simulink model "WBR_Simulator"  (R2023b)
settings: Solver=FixedStepAuto  StartTime=0.0  StopTime=60  FixedStep=0.001  MaxStep=0.001
undefined symbols (not defined in the file or in its folder): DiscIntNeverNeededParam, magnitude, robot_stats, SIMPARAM, X, Y, Z
libraries: sm_lib x73, nesl_utility x50, simulink x17, slpidlib x6, dsparch4 x2
(part 2 of 7)

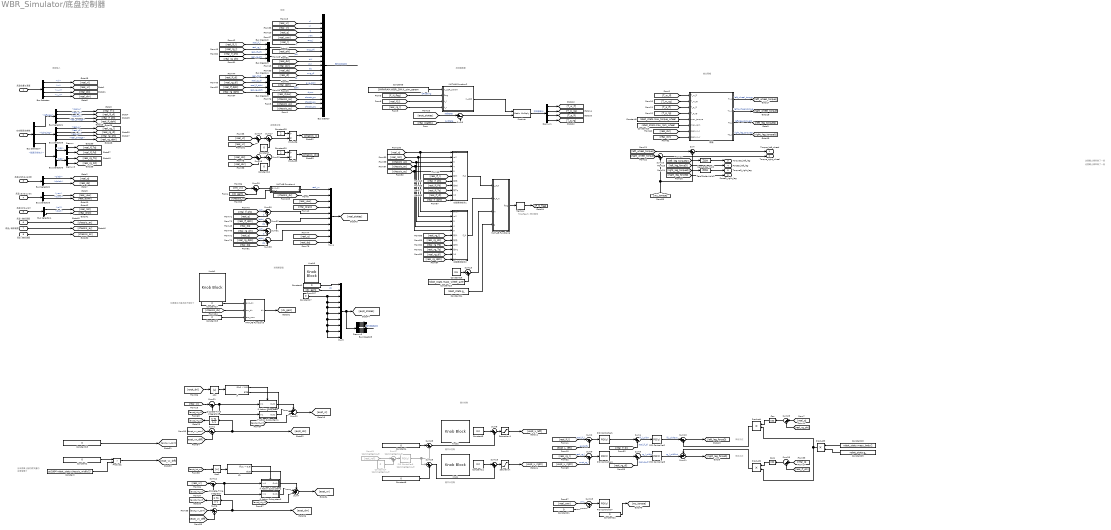
== system WBR_Simulator/底盘控制器 ==
  note: 参数输入
  note: F_N_flag为1表示离地
  note: 加速度过大基本就不受控了
  note: 应该再算上腿的劈叉量的
      | 这里偷懒了
  note: 腿齐长控制
  note: 伸出为正
  note: 伸出为正
  note: 这里截止频率除了一倍
  note: 这里截止频率除了一倍
  note: 腿齐长控制
  note: 装载真实值
  note: 装载期望值
  note: 观测
  note: 腿长控制
  note: 控制器解算
  note: 输出限幅
  底盘位置&速度 : Inport
  左右腿姿态参数 : Inport  Port=2
  底盘pitch&wpitch : Inport  Port=3
  底盘yaw&wyaw : Inport  Port=4
  底盘roll&wroll : Inport  Port=5
  底盘x轴加速度 : Inport  Port=6
  底盘y轴加速度 : Inport  Port=7
  底盘z轴加速度 : Inport  Port=8
  Abs : Abs  SaturateOnIntegerOverflow=off
  Abs1 : Abs  SaturateOnIntegerOverflow=off
  Bus Creator : BusCreator  Inputs=19
  Bus Creator{2..5} (4 alike) : BusCreator  Inputs=2
  Bus Creator8 : BusCreator  Inputs=10
  Bus Selector : BusSelector  OutputSignals=xl,xr,v_xl,v_xr
  Bus Selector1 : BusSelector  OutputSignals=real_L,real_dl,real_phi,real_omega
  Bus Selector2 : BusSelector  OutputSignals=pitch,dpitch
  Bus Selector3 : BusSelector  OutputSignals=yaw,dyaw
  Bus Selector4 : BusSelector  OutputSignals=roll,droll
  Bus Selector5 : BusSelector  OutputSignals=real_L,real_dl,real_phi,real_omega
  Bus Selector6 : BusSelector  OutputSignals=左腿,右腿
  Bus Selector7 : BusSelector  OutputSignals=left_leg,right_leg,腿真实有效力
  Constant : Constant  Value=pi/180*(robot_stats.chassis_width/2)
  Constant{1..2,4,7,12,15,17,21..22} (9 alike) : Constant  Value=0
  Constant10 : Constant  Value=robot_stats.max_rpm_wheel
  Constant11 : Constant  Value=0.2
  Constant14 : Constant  Commented=on  Value=0
  Constant16 : Constant  Value=0.5
  Constant18 : Constant  Value=robot_stats.mass_body/2
  Constant{19..20,27..28} (4 alike) : Constant  Value=2
  Constant23 : Constant  Value=robot_stats.mass_wheel_aver
  Constant24 : Constant  Value=robot_stats.g_
  Constant25 : Constant  Value=robot_stats.g_
  Constant3 : Constant  Value=0.2
  Constant5 : Constant  Value=SIMPARAM.WBR_SIM.K_sim_param
  Constant8 : Constant  Value=0  VectorParams1D=off
  Constant9 : Constant  Value=robot_stats.max_torque_wheel
  Cos : Trigonometry  Operator=cos
  Cos1 : Trigonometry  Operator=cos
  Demux : Demux  Outputs=2
  Demux1 : Demux
  Demux3 : Demux  Outputs=2
  Demux6 : Demux  Outputs=10
  Discrete-Time Integrator : DiscreteIntegrator  SampleTime=-1  ICPrevOutput=DiscIntNeverNeededParam  ICPrevScaledInput=DiscIntNeverNeededParam
  Discrete-Time Integrator1 : DiscreteIntegrator  SampleTime=-1  ICPrevOutput=DiscIntNeverNeededParam  ICPrevScaledInput=DiscIntNeverNeededParam
  From61 : From  Commented=on  GotoTag=real_roll
  If : If  IfExpression=u1 < 0.5
  If Action Subsystem : Subsystem  TreatAsAtomicUnit=on
  If Action Subsystem1 : Subsystem  TreatAsAtomicUnit=on
  If Action Subsystem2 : Subsystem  TreatAsAtomicUnit=on
  If Action Subsystem3 : Subsystem  TreatAsAtomicUnit=on
  If1 : If  IfExpression=u1 < 0.5
  Knob : KnobBlock  ScaleMin=-1  ScaleMax=1
  Knob1 : KnobBlock
  Knob2 : KnobBlock  ScaleMin=-1  ScaleMax=1
  Knob3 : KnobBlock
  MATLAB Function2 : MATLAB Function  TreatAsAtomicUnit=on
  MATLAB Function4 : MATLAB Function  TreatAsAtomicUnit=on
  MATLAB Function5 : MATLAB Function  TreatAsAtomicUnit=on
  MATLAB Function6 : MATLAB Function  TreatAsAtomicUnit=on
  Memory : Memory
  Mux4 : Mux  Inputs=10
  Mux5 : Mux  Inputs=10
  PID Controller1 : slpidlib/PID Controller  Controller=PID  Form=Parallel  TimeDomain=Discrete-time  UseExternalTs=off  SampleTime=-1  IntegratorMethod=Forward Euler  FilterMethod=Forward Euler  ControllerParametersSource=internal  P=8  I=0  UseKiTs=on  D=0.1  N=200  UseFilter=on  TunerSelectOption=Transfer Function Based (PID Tuner App)  InitialConditionSource=internal  InitialConditionForIntegrator=0  InitialConditionForFilter=0  DifferentiatorICPrevScaledInput=0  ExternalReset=none  TrackingMode=off  Kt=1  LimitOutput=off  SatLimitsSource=internal  UpperSaturationLimit=inf  LowerSaturationLimit=-inf  LinearizeAsGain=on  AntiWindupMode=none  Kb=1  LimitIntegrator=off  UpperIntegratorSaturationLimit=inf  LowerIntegratorSaturationLimit=-inf  POutMin=[]  POutMax=[]  IOutMin=[]  IOutMax=[]  DOutMin=[]  DOutMax=[]  NOutMin=[]  NOutMax=[]  SumOutMin=[]  SumOutMax=[]  SaturationOutMin=[]  SaturationOutMax=[]  PParamMin=[]  PParamMax=[]  IParamMin=[]  IParamMax=[]  DParamMin=[]  DParamMax=[]  NParamMin=[]  NParamMax=[]  KbParamMin=[]  KbParamMax=[]  KtParamMin=[]  KtParamMax=[]  KbOutMin=[]  KbOutMax=[]  KtOutMin=[]  KtOutMax=[]  IntegratorOutMin=[]  IntegratorOutMax=[]  FilterOutMin=[]  FilterOutMax=[]  SumI1OutMin=[]  SumI1OutMax=[]  SumI2OutMin=[]  SumI2OutMax=[]  SumI3OutMin=[]  SumI3OutMax=[]  SumI4OutMin=[]  SumI4OutMax=[]  SumDOutMin=[]  SumDOutMax=[]  DifferentiatorOutMin=[]  DifferentiatorOutMax=[]  FilterDiffOutCoefMin=[]  FilterDiffOutCoefMax=[]  ReciprocalOutMin=[]  ReciprocalOutMax=[]  SumDenOutMin=[]  SumDenOutMax=[]  SumNumOutMin=[]  SumNumOutMax=[]  DivideOutMin=[]  DivideOutMax=[]  UdiffTsProdOutMin=[]  UdiffTsProdOutMax=[]  NTsProdOutMin=[]  NTsProdOutMax=[]  UintegralTsProdOutMin=[]  UintegralTsProdOutMax=[]  UngainTsProdOutMin=[]  UngainTsProdOutMax=[]  ClampingZeroOutDataTypeStr=Inherit: Inherit via back propagation  ClampingZeroOutMin=[]  ClampingZeroOutMax=[]  FilterDenConstantOutDataTypeStr=Inherit: Inherit via back propagation  FilterDenConstantOutMin=[]  FilterDenConstantOutMax=[]  PCopyOutDataTypeStr=Inherit: Inherit via back propagation  PCopyOutMin=[]  PCopyOutMax=[]  NCopyOutDataTypeStr=Inherit: Inherit via back propagation  NCopyOutMin=[]  NCopyOutMax=[]  IntegratorContinuousStateAttributes=''  IntegratorStateMustResolveToSignalObject=off  IntegratorRTWStateStorageClass=Auto  FilterContinuousStateAttributes=''  FilterStateMustResolveToSignalObject=off  FilterRTWStateStorageClass=Auto  ParallelPVariant=InternalParameters  IdealPVariant=Disabled  IVariant=InternalParameters  DVariant=InternalParameters  IntegratorVariant=Discrete  SatVariant=Disabled  AWVariant=Passthrough  PCopyVariant=Disabled  TRVariant=Disabled  FdbkBlocksVariant=Forward  IdealPFdbkVariant=Disabled  SatFdbkVariant=Disabled  DerivativeFilterVariant=ForwardEulerFilter  NVariant=InternalParameters  NCopyVariant=Disabled  FilterICVariant=InternalICsFilter  IntegratorICVariant=InternalICs  ExternalResetVariant=Disabled  TRSumVariant=Passthrough  SumFdbkVariant=Disabled  SumVariant=Sum_PID  TsampFilterVariant=InternalTs  TsampNgainVariant=Passthrough  TsampIntegralVariant=Disabled_SignalSpec  ExternalSaturationOutDataTypeStr=Inherit: Same as second input
  PID Controller2 : slpidlib/PID Controller  Controller=PID  Form=Parallel  TimeDomain=Discrete-time  UseExternalTs=off  SampleTime=-1  IntegratorMethod=Forward Euler  FilterMethod=Forward Euler  ControllerParametersSource=internal  P=50  I=0  UseKiTs=off  D=0.1  N=100  UseFilter=on  TunerSelectOption=Transfer Function Based (PID Tuner App)  InitialConditionSource=internal  InitialConditionForIntegrator=0  InitialConditionForFilter=0  DifferentiatorICPrevScaledInput=0  ExternalReset=none  TrackingMode=off  Kt=1  LimitOutput=off  SatLimitsSource=internal  UpperSaturationLimit=800  LowerSaturationLimit=-800  LinearizeAsGain=on  AntiWindupMode=none  Kb=1  LimitIntegrator=off  UpperIntegratorSaturationLimit=inf  LowerIntegratorSaturationLimit=-inf  POutMin=[]  POutMax=[]  IOutMin=[]  IOutMax=[]  DOutMin=[]  DOutMax=[]  NOutMin=[]  NOutMax=[]  SumOutMin=[]  SumOutMax=[]  SaturationOutMin=[]  SaturationOutMax=[]  PParamMin=[]  PParamMax=[]  IParamMin=[]  IParamMax=[]  DParamMin=[]  DParamMax=[]  NParamMin=[]  NParamMax=[]  KbParamMin=[]  KbParamMax=[]  KtParamMin=[]  KtParamMax=[]  KbOutMin=[]  KbOutMax=[]  KtOutMin=[]  KtOutMax=[]  IntegratorOutMin=[]  IntegratorOutMax=[]  FilterOutMin=[]  FilterOutMax=[]  SumI1OutMin=[]  SumI1OutMax=[]  SumI2OutMin=[]  SumI2OutMax=[]  SumI3OutMin=[]  SumI3OutMax=[]  SumI4OutMin=[]  SumI4OutMax=[]  SumDOutMin=[]  SumDOutMax=[]  DifferentiatorOutMin=[]  DifferentiatorOutMax=[]  FilterDiffOutCoefMin=[]  FilterDiffOutCoefMax=[]  ReciprocalOutMin=[]  ReciprocalOutMax=[]  SumDenOutMin=[]  SumDenOutMax=[]  SumNumOutMin=[]  SumNumOutMax=[]  DivideOutMin=[]  DivideOutMax=[]  UdiffTsProdOutMin=[]  UdiffTsProdOutMax=[]  NTsProdOutMin=[]  NTsProdOutMax=[]  UintegralTsProdOutMin=[]  UintegralTsProdOutMax=[]  UngainTsProdOutMin=[]  UngainTsProdOutMax=[]  ClampingZeroOutDataTypeStr=Inherit: Inherit via back propagation  ClampingZeroOutMin=[]  ClampingZeroOutMax=[]  FilterDenConstantOutDataTypeStr=Inherit: Inherit via back propagation  FilterDenConstantOutMin=[]  FilterDenConstantOutMax=[]  PCopyOutDataTypeStr=Inherit: Inherit via back propagation  PCopyOutMin=[]  PCopyOutMax=[]  NCopyOutDataTypeStr=Inherit: Inherit via back propagation  NCopyOutMin=[]  NCopyOutMax=[]  IntegratorContinuousStateAttributes=''  IntegratorStateMustResolveToSignalObject=off  IntegratorRTWStateStorageClass=Auto  FilterContinuousStateAttributes=''  FilterStateMustResolveToSignalObject=off  FilterRTWStateStorageClass=Auto  ParallelPVariant=InternalParameters  IdealPVariant=Disabled  IVariant=InternalParameters  DVariant=InternalParameters  IntegratorVariant=Discrete  SatVariant=Disabled  AWVariant=Passthrough  PCopyVariant=Disabled  TRVariant=Disabled  FdbkBlocksVariant=Forward  IdealPFdbkVariant=Disabled  SatFdbkVariant=Disabled  DerivativeFilterVariant=ForwardEulerFilter  NVariant=InternalParameters  NCopyVariant=Disabled  FilterICVariant=InternalICsFilter  IntegratorICVariant=InternalICs  ExternalResetVariant=Disabled  TRSumVariant=Passthrough  SumFdbkVariant=Disabled  SumVariant=Sum_PID  TsampFilterVariant=InternalTs  TsampNgainVariant=Passthrough  TsampIntegralVariant=Disabled_SignalSpec  ExternalSaturationOutDataTypeStr=Inherit: Same as second input
  PID Controller3 : slpidlib/PID Controller  Controller=PID  Form=Parallel  TimeDomain=Discrete-time  UseExternalTs=off  SampleTime=-1  IntegratorMethod=Forward Euler  FilterMethod=Forward Euler  ControllerParametersSource=internal  P=50  I=0  UseKiTs=off  D=0.1  N=100  UseFilter=on  TunerSelectOption=Transfer Function Based (PID Tuner App)  InitialConditionSource=internal  InitialConditionForIntegrator=0  InitialConditionForFilter=0  DifferentiatorICPrevScaledInput=0  ExternalReset=none  TrackingMode=off  Kt=1  LimitOutput=off  SatLimitsSource=internal  UpperSaturationLimit=800  LowerSaturationLimit=-800  LinearizeAsGain=on  AntiWindupMode=none  Kb=1  LimitIntegrator=off  UpperIntegratorSaturationLimit=inf  LowerIntegratorSaturationLimit=-inf  POutMin=[]  POutMax=[]  IOutMin=[]  IOutMax=[]  DOutMin=[]  DOutMax=[]  NOutMin=[]  NOutMax=[]  SumOutMin=[]  SumOutMax=[]  SaturationOutMin=[]  SaturationOutMax=[]  PParamMin=[]  PParamMax=[]  IParamMin=[]  IParamMax=[]  DParamMin=[]  DParamMax=[]  NParamMin=[]  NParamMax=[]  KbParamMin=[]  KbParamMax=[]  KtParamMin=[]  KtParamMax=[]  KbOutMin=[]  KbOutMax=[]  KtOutMin=[]  KtOutMax=[]  IntegratorOutMin=[]  IntegratorOutMax=[]  FilterOutMin=[]  FilterOutMax=[]  SumI1OutMin=[]  SumI1OutMax=[]  SumI2OutMin=[]  SumI2OutMax=[]  SumI3OutMin=[]  SumI3OutMax=[]  SumI4OutMin=[]  SumI4OutMax=[]  SumDOutMin=[]  SumDOutMax=[]  DifferentiatorOutMin=[]  DifferentiatorOutMax=[]  FilterDiffOutCoefMin=[]  FilterDiffOutCoefMax=[]  ReciprocalOutMin=[]  ReciprocalOutMax=[]  SumDenOutMin=[]  SumDenOutMax=[]  SumNumOutMin=[]  SumNumOutMax=[]  DivideOutMin=[]  DivideOutMax=[]  UdiffTsProdOutMin=[]  UdiffTsProdOutMax=[]  NTsProdOutMin=[]  NTsProdOutMax=[]  UintegralTsProdOutMin=[]  UintegralTsProdOutMax=[]  UngainTsProdOutMin=[]  UngainTsProdOutMax=[]  ClampingZeroOutDataTypeStr=Inherit: Inherit via back propagation  ClampingZeroOutMin=[]  ClampingZeroOutMax=[]  FilterDenConstantOutDataTypeStr=Inherit: Inherit via back propagation  FilterDenConstantOutMin=[]  FilterDenConstantOutMax=[]  PCopyOutDataTypeStr=Inherit: Inherit via back propagation  PCopyOutMin=[]  PCopyOutMax=[]  NCopyOutDataTypeStr=Inherit: Inherit via back propagation  NCopyOutMin=[]  NCopyOutMax=[]  IntegratorContinuousStateAttributes=''  IntegratorStateMustResolveToSignalObject=off  IntegratorRTWStateStorageClass=Auto  FilterContinuousStateAttributes=''  FilterStateMustResolveToSignalObject=off  FilterRTWStateStorageClass=Auto  ParallelPVariant=InternalParameters  IdealPVariant=Disabled  IVariant=InternalParameters  DVariant=InternalParameters  IntegratorVariant=Discrete  SatVariant=Disabled  AWVariant=Passthrough  PCopyVariant=Disabled  TRVariant=Disabled  FdbkBlocksVariant=Forward  IdealPFdbkVariant=Disabled  SatFdbkVariant=Disabled  DerivativeFilterVariant=ForwardEulerFilter  NVariant=InternalParameters  NCopyVariant=Disabled  FilterICVariant=InternalICsFilter  IntegratorICVariant=InternalICs  ExternalResetVariant=Disabled  TRSumVariant=Passthrough  SumFdbkVariant=Disabled  SumVariant=Sum_PID  TsampFilterVariant=InternalTs  TsampNgainVariant=Passthrough  TsampIntegralVariant=Disabled_SignalSpec  ExternalSaturationOutDataTypeStr=Inherit: Same as second input
  PID Controller4 : slpidlib/PID Controller  Controller=PID  Form=Parallel  TimeDomain=Discrete-time  UseExternalTs=off  SampleTime=-1  IntegratorMethod=Forward Euler  FilterMethod=Forward Euler  ControllerParametersSource=internal  P=8  I=0  UseKiTs=on  D=0.1  N=200  UseFilter=on  TunerSelectOption=Transfer Function Based (PID Tuner App)  InitialConditionSource=internal  InitialConditionForIntegrator=0  InitialConditionForFilter=0  DifferentiatorICPrevScaledInput=0  ExternalReset=none  TrackingMode=off  Kt=1  LimitOutput=off  SatLimitsSource=internal  UpperSaturationLimit=inf  LowerSaturationLimit=-inf  LinearizeAsGain=on  AntiWindupMode=none  Kb=1  LimitIntegrator=off  UpperIntegratorSaturationLimit=inf  LowerIntegratorSaturationLimit=-inf  POutMin=[]  POutMax=[]  IOutMin=[]  IOutMax=[]  DOutMin=[]  DOutMax=[]  NOutMin=[]  NOutMax=[]  SumOutMin=[]  SumOutMax=[]  SaturationOutMin=[]  SaturationOutMax=[]  PParamMin=[]  PParamMax=[]  IParamMin=[]  IParamMax=[]  DParamMin=[]  DParamMax=[]  NParamMin=[]  NParamMax=[]  KbParamMin=[]  KbParamMax=[]  KtParamMin=[]  KtParamMax=[]  KbOutMin=[]  KbOutMax=[]  KtOutMin=[]  KtOutMax=[]  IntegratorOutMin=[]  IntegratorOutMax=[]  FilterOutMin=[]  FilterOutMax=[]  SumI1OutMin=[]  SumI1OutMax=[]  SumI2OutMin=[]  SumI2OutMax=[]  SumI3OutMin=[]  SumI3OutMax=[]  SumI4OutMin=[]  SumI4OutMax=[]  SumDOutMin=[]  SumDOutMax=[]  DifferentiatorOutMin=[]  DifferentiatorOutMax=[]  FilterDiffOutCoefMin=[]  FilterDiffOutCoefMax=[]  ReciprocalOutMin=[]  ReciprocalOutMax=[]  SumDenOutMin=[]  SumDenOutMax=[]  SumNumOutMin=[]  SumNumOutMax=[]  DivideOutMin=[]  DivideOutMax=[]  UdiffTsProdOutMin=[]  UdiffTsProdOutMax=[]  NTsProdOutMin=[]  NTsProdOutMax=[]  UintegralTsProdOutMin=[]  UintegralTsProdOutMax=[]  UngainTsProdOutMin=[]  UngainTsProdOutMax=[]  ClampingZeroOutDataTypeStr=Inherit: Inherit via back propagation  ClampingZeroOutMin=[]  ClampingZeroOutMax=[]  FilterDenConstantOutDataTypeStr=Inherit: Inherit via back propagation  FilterDenConstantOutMin=[]  FilterDenConstantOutMax=[]  PCopyOutDataTypeStr=Inherit: Inherit via back propagation  PCopyOutMin=[]  PCopyOutMax=[]  NCopyOutDataTypeStr=Inherit: Inherit via back propagation  NCopyOutMin=[]  NCopyOutMax=[]  IntegratorContinuousStateAttributes=''  IntegratorStateMustResolveToSignalObject=off  IntegratorRTWStateStorageClass=Auto  FilterContinuousStateAttributes=''  FilterStateMustResolveToSignalObject=off  FilterRTWStateStorageClass=Auto  ParallelPVariant=InternalParameters  IdealPVariant=Disabled  IVariant=InternalParameters  DVariant=InternalParameters  IntegratorVariant=Discrete  SatVariant=Disabled  AWVariant=Passthrough  PCopyVariant=Disabled  TRVariant=Disabled  FdbkBlocksVariant=Forward  IdealPFdbkVariant=Disabled  SatFdbkVariant=Disabled  DerivativeFilterVariant=ForwardEulerFilter  NVariant=InternalParameters  NCopyVariant=Disabled  FilterICVariant=InternalICsFilter  IntegratorICVariant=InternalICs  ExternalResetVariant=Disabled  TRSumVariant=Passthrough  SumFdbkVariant=Disabled  SumVariant=Sum_PID  TsampFilterVariant=InternalTs  TsampNgainVariant=Passthrough  TsampIntegralVariant=Disabled_SignalSpec  ExternalSaturationOutDataTypeStr=Inherit: Same as second input
  PID Controller7 : slpidlib/PID Controller  Controller=PID  Form=Parallel  TimeDomain=Discrete-time  UseExternalTs=off  SampleTime=-1  IntegratorMethod=Forward Euler  FilterMethod=Forward Euler  ControllerParametersSource=internal  P=4  I=5  UseKiTs=on  D=0.001  N=200  UseFilter=on  TunerSelectOption=Transfer Function Based (PID Tuner App)  InitialConditionSource=internal  InitialConditionForIntegrator=0  InitialConditionForFilter=0  DifferentiatorICPrevScaledInput=0  ExternalReset=none  TrackingMode=off  Kt=1  LimitOutput=off  SatLimitsSource=internal  UpperSaturationLimit=inf  LowerSaturationLimit=-inf  LinearizeAsGain=on  AntiWindupMode=none  Kb=1  LimitIntegrator=off  UpperIntegratorSaturationLimit=inf  LowerIntegratorSaturationLimit=-inf  POutMin=[]  POutMax=[]  IOutMin=[]  IOutMax=[]  DOutMin=[]  DOutMax=[]  NOutMin=[]  NOutMax=[]  SumOutMin=[]  SumOutMax=[]  SaturationOutMin=[]  SaturationOutMax=[]  PParamMin=[]  PParamMax=[]  IParamMin=[]  IParamMax=[]  DParamMin=[]  DParamMax=[]  NParamMin=[]  NParamMax=[]  KbParamMin=[]  KbParamMax=[]  KtParamMin=[]  KtParamMax=[]  KbOutMin=[]  KbOutMax=[]  KtOutMin=[]  KtOutMax=[]  IntegratorOutMin=[]  IntegratorOutMax=[]  FilterOutMin=[]  FilterOutMax=[]  SumI1OutMin=[]  SumI1OutMax=[]  SumI2OutMin=[]  SumI2OutMax=[]  SumI3OutMin=[]  SumI3OutMax=[]  SumI4OutMin=[]  SumI4OutMax=[]  SumDOutMin=[]  SumDOutMax=[]  DifferentiatorOutMin=[]  DifferentiatorOutMax=[]  FilterDiffOutCoefMin=[]  FilterDiffOutCoefMax=[]  ReciprocalOutMin=[]  ReciprocalOutMax=[]  SumDenOutMin=[]  SumDenOutMax=[]  SumNumOutMin=[]  SumNumOutMax=[]  DivideOutMin=[]  DivideOutMax=[]  UdiffTsProdOutMin=[]  UdiffTsProdOutMax=[]  NTsProdOutMin=[]  NTsProdOutMax=[]  UintegralTsProdOutMin=[]  UintegralTsProdOutMax=[]  UngainTsProdOutMin=[]  UngainTsProdOutMax=[]  ClampingZeroOutDataTypeStr=Inherit: Inherit via back propagation  ClampingZeroOutMin=[]  ClampingZeroOutMax=[]  FilterDenConstantOutDataTypeStr=Inherit: Inherit via back propagation  FilterDenConstantOutMin=[]  FilterDenConstantOutMax=[]  PCopyOutDataTypeStr=Inherit: Inherit via back propagation  PCopyOutMin=[]  PCopyOutMax=[]  NCopyOutDataTypeStr=Inherit: Inherit via back propagation  NCopyOutMin=[]  NCopyOutMax=[]  IntegratorContinuousStateAttributes=''  IntegratorStateMustResolveToSignalObject=off  IntegratorRTWStateStorageClass=Auto  FilterContinuousStateAttributes=''  FilterStateMustResolveToSignalObject=off  FilterRTWStateStorageClass=Auto  ParallelPVariant=InternalParameters  IdealPVariant=Disabled  IVariant=InternalParameters  DVariant=InternalParameters  IntegratorVariant=Discrete  SatVariant=Disabled  AWVariant=Passthrough  PCopyVariant=Disabled  TRVariant=Disabled  FdbkBlocksVariant=Forward  IdealPFdbkVariant=Disabled  SatFdbkVariant=Disabled  DerivativeFilterVariant=ForwardEulerFilter  NVariant=InternalParameters  NCopyVariant=Disabled  FilterICVariant=InternalICsFilter  IntegratorICVariant=InternalICs  ExternalResetVariant=Disabled  TRSumVariant=Passthrough  SumFdbkVariant=Disabled  SumVariant=Sum_PID  TsampFilterVariant=InternalTs  TsampNgainVariant=Passthrough  TsampIntegralVariant=Disabled_SignalSpec  ExternalSaturationOutDataTypeStr=Inherit: Same as second input
  PID Controller9 : slpidlib/PID Controller  Commented=on  Controller=PID  Form=Parallel  TimeDomain=Discrete-time  UseExternalTs=off  SampleTime=-1  IntegratorMethod=Forward Euler  FilterMethod=Forward Euler  ControllerParametersSource=internal  P=8  I=5  UseKiTs=on  D=0.1  N=200  UseFilter=on  TunerSelectOption=Transfer Function Based (PID Tuner App)  InitialConditionSource=internal  InitialConditionForIntegrator=0  InitialConditionForFilter=0  DifferentiatorICPrevScaledInput=0  ExternalReset=none  TrackingMode=off  Kt=1  LimitOutput=off  SatLimitsSource=internal  UpperSaturationLimit=inf  LowerSaturationLimit=-inf  LinearizeAsGain=on  AntiWindupMode=none  Kb=1  LimitIntegrator=off  UpperIntegratorSaturationLimit=inf  LowerIntegratorSaturationLimit=-inf  POutMin=[]  POutMax=[]  IOutMin=[]  IOutMax=[]  DOutMin=[]  DOutMax=[]  NOutMin=[]  NOutMax=[]  SumOutMin=[]  SumOutMax=[]  SaturationOutMin=[]  SaturationOutMax=[]  PParamMin=[]  PParamMax=[]  IParamMin=[]  IParamMax=[]  DParamMin=[]  DParamMax=[]  NParamMin=[]  NParamMax=[]  KbParamMin=[]  KbParamMax=[]  KtParamMin=[]  KtParamMax=[]  KbOutMin=[]  KbOutMax=[]  KtOutMin=[]  KtOutMax=[]  IntegratorOutMin=[]  IntegratorOutMax=[]  FilterOutMin=[]  FilterOutMax=[]  SumI1OutMin=[]  SumI1OutMax=[]  SumI2OutMin=[]  SumI2OutMax=[]  SumI3OutMin=[]  SumI3OutMax=[]  SumI4OutMin=[]  SumI4OutMax=[]  SumDOutMin=[]  SumDOutMax=[]  DifferentiatorOutMin=[]  DifferentiatorOutMax=[]  FilterDiffOutCoefMin=[]  FilterDiffOutCoefMax=[]  ReciprocalOutMin=[]  ReciprocalOutMax=[]  SumDenOutMin=[]  SumDenOutMax=[]  SumNumOutMin=[]  SumNumOutMax=[]  DivideOutMin=[]  DivideOutMax=[]  UdiffTsProdOutMin=[]  UdiffTsProdOutMax=[]  NTsProdOutMin=[]  NTsProdOutMax=[]  UintegralTsProdOutMin=[]  UintegralTsProdOutMax=[]  UngainTsProdOutMin=[]  UngainTsProdOutMax=[]  ClampingZeroOutDataTypeStr=Inherit: Inherit via back propagation  ClampingZeroOutMin=[]  ClampingZeroOutMax=[]  FilterDenConstantOutDataTypeStr=Inherit: Inherit via back propagation  FilterDenConstantOutMin=[]  FilterDenConstantOutMax=[]  PCopyOutDataTypeStr=Inherit: Inherit via back propagation  PCopyOutMin=[]  PCopyOutMax=[]  NCopyOutDataTypeStr=Inherit: Inherit via back propagation  NCopyOutMin=[]  NCopyOutMax=[]  IntegratorContinuousStateAttributes=''  IntegratorStateMustResolveToSignalObject=off  IntegratorRTWStateStorageClass=Auto  FilterContinuousStateAttributes=''  FilterStateMustResolveToSignalObject=off  FilterRTWStateStorageClass=Auto  ParallelPVariant=InternalParameters  IdealPVariant=Disabled  IVariant=InternalParameters  DVariant=InternalParameters  IntegratorVariant=Discrete  SatVariant=Disabled  AWVariant=Passthrough  PCopyVariant=Disabled  TRVariant=Disabled  FdbkBlocksVariant=Forward  IdealPFdbkVariant=Disabled  SatFdbkVariant=Disabled  DerivativeFilterVariant=ForwardEulerFilter  NVariant=InternalParameters  NCopyVariant=Disabled  FilterICVariant=InternalICsFilter  IntegratorICVariant=InternalICs  ExternalResetVariant=Disabled  TRSumVariant=Passthrough  SumFdbkVariant=Disabled  SumVariant=Sum_PID  TsampFilterVariant=InternalTs  TsampNgainVariant=Passthrough  TsampIntegralVariant=Disabled_SignalSpec  ExternalSaturationOutDataTypeStr=Inherit: Same as second input
  Product : Product  Multiplication=Matrix(*)
  Product1 : Product
  Product2 : Product  Inputs=**
  Product3 : Product  Inputs=**
  Product4 : Product  Inputs=**
  Product5 : Product  Inputs=/*
  Product6 : Product  Inputs=/*
  Saturation : Saturate  UpperLimit=robot_stats.leg_length_max  LowerLimit=robot_stats.leg_length_min
  Saturation1 : Saturate  UpperLimit=robot_stats.leg_length_max  LowerLimit=robot_stats.leg_length_min
  Sum{,1,3..5,25..26,28} (8 alike) : Sum  Inputs=|+-
  Sum{6,8,10,13,16..20,23..24,29..33} (16 alike) : Sum  Inputs=|++
  Sum11 : Sum  Inputs=++|
  Sum{2,9,12,15,21} (5 alike) : Sum  Inputs=|-+
  Sum22 : Sum  Inputs=--+|
  Sum27 : Sum  Commented=on  Inputs=|-+
  Sum7 : Sum  Inputs=--+|
  Zero-Order Hold : ZeroOrderHold  SampleTime=0.001
  Zero-Order Hold2 : ZeroOrderHold  SampleTime=0.001
  左腿离地检测1 : Subsystem
  左腿离地检测2 : Subsystem
  限幅 : MATLAB Function  TreatAsAtomicUnit=on
  Torque_left_wheel : Outport
  Torque_right_wheel : Outport  Port=2
  TorqueQ_left_leg : Outport  Port=3
  ForceD_left_leg : Outport  Port=4
  TorqueQ_right_leg : Outport  Port=5
  ForceD_right_leg : Outport  Port=6
  wires:
  [real_states] -> Sum3/2  "curState"
  限幅/1(Tx_l) -> [left_wheel_torque]  "left_wheel_torque"
  Product/1 -> Demux1/1  "控制器输出"
  [expt_states] -> Sum3/1  "refState"
  限幅/3(Tq_l) -> [left_leg_torqueQ]  "left_leg_torqueQ"
  [real_lf_l] -> Sum2/1  "real_lf_l"
  Sum2/1 -> PID Controller1/1
  Constant10/1 -> 限幅/6(max_rpm)
  [real_dxl] -> 限幅/7(real_vx_l)
  Constant9/1 -> 限幅/5(max_torque)
  限幅/2(Tx_r) -> [right_wheel_torque]  "right_wheel_torque"
  PID Controller1/1 -> Sum4/1
  Sum3/1 -> Product/2
  限幅/4(Tq_r) -> [right_leg_torqueQ]  "right_leg_torqueQ"
  Bus Selector7/2 -> Bus Selector5/1  "<right_leg>"
  底盘yaw&wyaw/1 -> Bus Selector3/1
  Bus Selector7/1 -> Bus Selector1/1  "<left_leg>"
  底盘pitch&wpitch/1 -> Bus Selector2/1
  Bus Selector/2 -> [real_xr]  "<xr>"
  Bus Selector3/1 -> [real_yaw]  "<yaw>"
  Bus Selector1/1 -> [real_lf_l]  "<real_L>"
  Bus Selector1/3 -> [real_lf_phi]  "<real_phi>"
  Bus Selector5/1 -> [real_rg_l]  "<real_L>"
  Bus Selector5/3 -> [real_rg_phi]  "<real_phi>"
  [real_rg_l] -> Sum9/1  "real_rg_l"
  Sum9/1 -> PID Controller4/1
  PID Controller4/1 -> Sum5/1
  Bus Creator/1 -> ?  "整车实际姿态"
  [real_lf_l] -> Bus Creator2/1  "real_lf_l"
  [real_rg_l] -> Bus Creator2/2  "real_rg_l"
  [real_lf_phi] -> Bus Creator3/1  "real_lf_phi"
  [real_lf_dl] -> Bus Creator4/1  "real_lf_dl"
  [real_rg_dl] -> Bus Creator4/2  "real_rg_dl"
  [real_lf_dphi] -> Bus Creator5/1  "real_lf_dphi"
  [real_rg_dphi] -> Bus Creator5/2  "real_rg_dphi"
  [real_dphi] -> Bus Creator/14  "avg_dphi"
  Bus Creator5/1 -> Bus Creator/15  "dphi"
  [real_dyaw] -> Bus Creator/16  "dyaw"
  Bus Creator4/1 -> Bus Creator/13  "dl"
  [real_dl] -> Bus Creator/12  "avg_dl"
  [real_dq] -> Bus Creator/11  "dq"
  [real_dxl] -> Bus Creator/9  "dxl"
  Bus Creator3/1 -> Bus Creator/8  "phi"
  [real_phi] -> Bus Creator/7  "avg_phi"
  Bus Creator2/1 -> Bus Creator/6  "l"
  [real_l] -> Bus Creator/5  "avg_l"
  [real_yaw] -> Bus Creator/4  "yaw"
  [real_q] -> Bus Creator/3  "q"
  [real_rg_dl] -> Sum5/2  "real_rg_dl"
  [real_lf_dl] -> Sum4/2  "real_lf_dl"
  Sum5/1 -> PID Controller3/1  "rg_l_pidIn"
  Sum4/1 -> PID Controller2/1  "lf_l_pidIn"
  Demux1/2 -> [T_w_rg]
  Demux1/3 -> [T_p_lf]
  Constant11/1 -> Sum19/1
  [expt_L_left] -> Sum2/2  "expt_lf_l"
  [expt_L_right] -> Sum9/2  "expt_rg_l"
  Sum19/1 -> Saturation/1
  Saturation/1 -> [expt_L_right]
  Bus Selector/1 -> [real_xl]  "<xl>"
  [real_xr] -> Bus Creator/2  "xr"
  [real_xl] -> Bus Creator/1  "xl"
  Demux1/1 -> [T_w_lf]
  [T_w_lf] -> 限幅/1(T_w_lf)
  [T_w_rg] -> 限幅/2(T_w_rg)
  [T_p_lf] -> 限幅/3(T_p_lf)
  [T_p_rg] -> 限幅/4(T_p_rg)
  Demux1/4 -> [T_p_rg]
  [real_dxr] -> Bus Creator/10  "dxr"
  [expt_int_xl] -> Sum21/2
  [real_xl] -> Sum21/1
  Constant/1 -> Product1/2
  Constant2/1 -> Product1/1
  Discrete-Time Integrator/1 -> [expt_int_xr]
  [expt_int_xr] -> Sum12/2
  [real_xr] -> Sum12/1
  [expt_vx_diff] -> Sum1/2
  [expt_vx_com] -> Sum1/1
  Sum1/1 -> Discrete-Time Integrator1/1, [expt_dxl]
  [expt_vx_com] -> Sum6/1
  [expt_vx_diff] -> Sum6/2
  Sum6/1 -> Discrete-Time Integrator/1, [expt_dxr]
  底盘位置&速度/1 -> Bus Selector/1
  左右腿姿态参数/1 -> Bus Selector7/1
  Bus Selector/3 -> [real_dxl]  "<v_xl>"
  Bus Selector/4 -> [real_dxr]  "<v_xr>"
  Bus Selector1/2 -> [real_lf_dl]  "<real_dl>"
  Bus Selector1/4 -> [real_lf_dphi]  "<real_omega>"
  Bus Selector5/2 -> [real_rg_dl]  "<real_dl>"
  Bus Selector5/4 -> [real_rg_dphi]  "<real_omega>"
  [right_leg_torqueQ] -> Zero-Order Hold2/1
  [left_leg_torqueQ] -> Zero-Order Hold/1
  Bus Selector3/2 -> [real_dyaw]  "<dyaw>"
  Sum22/1 -> [expt_xl]
  Product1/1 -> [expt_vx_diff]
  Constant15/1 -> [expt_vx_com]
  [expt_dxl] -> Abs/1
  Abs/1 -> If/1
  If/1 -> If Action Subsystem/Action
  If Action Subsystem/1(Out1) -> Sum22/1
  If/2 -> If Action Subsystem1/Action
  Sum21/1 -> If Action Subsystem1/1(In1), If Action Subsystem/1(In1)
  If Action Subsystem1/1(Out1) -> Sum22/2
  [expt_int_xl] -> Sum22/3
  If Action Subsystem2/1(Out1) -> Sum7/1
  If Action Subsystem3/1(Out1) -> Sum7/2
  Sum12/1 -> If Action Subsystem3/1(In1), If Action Subsystem2/1(In1)
  If1/2 -> If Action Subsystem3/Action
  [expt_int_xl] -> Sum7/3
  If1/1 -> If Action Subsystem2/Action
  [expt_int_xr] -> Abs1/1
  Sum7/1 -> [expt_xr]
  Abs1/1 -> If1/1
  [real_dxr] -> 限幅/8(real_vx_r)
  Sum8/1 -> Saturation1/1
  Constant3/1 -> Sum8/1
  Saturation1/1 -> [expt_L_left]
  PID Controller2/1 -> Sum10/1  "lf_l_pidOut"
  PID Controller3/1 -> Sum11/2  "rg_l_pidOut"
  Product4/1 -> Sum10/2
  Constant5/1 -> MATLAB Function2/1(K_LQR_param)
  Bus Selector7/3 -> Bus Selector6/1  "<腿真实有效力>"
  Bus Selector6/1 -> Demux/1  "<左腿>"
  Bus Selector6/2 -> Demux3/1  "<右腿>"
  Demux/2 -> [real_lf_Fd]
  Demux3/2 -> [real_rg_Fd]
  Demux/1 -> [real_lf_Tq]
  Demux3/1 -> [real_rg_Tq]
  MATLAB Function2/1(K_LQR) -> Product/1
  [real_lf_l] -> MATLAB Function2/3(L_l)
  [real_rg_l] -> MATLAB Function2/4(L_r)
  Mux4/1 -> [real_states]
  Bus Selector2/1 -> [real_q]  "<pitch>"
  Bus Selector2/2 -> [real_dq]  "<dpitch>"
  [real_yaw] -> Sum15/1  "yaw"
  Constant21/1 -> Sum15/2
  Sum15/1 -> PID Controller7/1
  [left_wheel_torque] -> Sum/1
  [wz_torque] -> Sum16/2, Sum/2
  [right_wheel_torque] -> Sum16/1
  底盘z轴加速度/1 -> [chassis_az]
  Constant20/1 -> Product5/1
  [real_dxr] -> Sum18/2
  [real_dxl] -> Sum18/1
  [init_vx] -> Sum20/1
  [dx_gain] -> Sum20/2
  Sum20/1 -> MATLAB Function4/1(exp_dx)
  [real_xl] -> Sum24/1
  [real_xr] -> Sum24/2
  Constant28/1 -> Product6/1
  Product6/1 -> [chassis_x]
  Product5/1 -> [chassis_dx]
  [chassis_x] -> MATLAB Function4/2(cur_x)
  Constant27/1 -> MATLAB Function5/1(exp_dx)
  [chassis_dx] -> MATLAB Function5/2(cur_dx)
  Constant19/1 -> MATLAB Function5/3(acc_max)
  MATLAB Function5/1(dx) -> [dx_gain]
  [real_rg_phi] -> 左腿离地检测2/7(腿角)
  [real_rg_l] -> 左腿离地检测2/6(腿长)
  [real_rg_dl] -> 左腿离地检测2/10(腿长变化率)
  [real_rg_dphi] -> 左腿离地检测2/11(腿角变化率)
  [real_rg_Fd] -> 左腿离地检测2/8(腿Fd)
  [real_rg_Tq] -> 左腿离地检测2/9(腿Tq)
  左腿离地检测2/1(F_N) -> MATLAB Function6/2(R_F_N)
  MATLAB Function6/1(flag) -> Memory/1
  [real_lf_Tq] -> 左腿离地检测1/9(腿Tq)
  [real_lf_l] -> 左腿离地检测1/6(腿长)
  [chassis_az] -> 左腿离地检测2/5(底盘z轴加速度), 左腿离地检测1/5(底盘z轴加速度)
  [real_lf_dl] -> 左腿离地检测1/10(腿长变化率)
  [real_lf_phi] -> 左腿离地检测1/7(腿角)
  [real_lf_Fd] -> 左腿离地检测1/8(腿Fd)
  [real_lf_dphi] -> 左腿离地检测1/11(腿角变化率)
  左腿离地检测1/1(F_N) -> MATLAB Function6/1(L_F_N)
  Constant24/1 -> MATLAB Function6/4(g)
  MATLAB Function4/1(y) -> Mux4/1  "real_xr"
  [chassis_dx] -> Mux4/2
  [real_dq] -> Mux4/10
  [real_q] -> Mux4/9
  [real_yaw] -> Mux4/3
  [real_dyaw] -> Mux4/4
  Constant17/1 -> Mux5/10, Mux5/9, Mux5/8, Mux5/7, Mux5/6, Mux5/5, Mux5/4, Mux5/3
  Mux5/1 -> Demux6/1, [expt_states]
  [dx_gain] -> Mux5/2  "ds"
  Demux6/4 -> Bus Creator8/4
  Demux6/8 -> Bus Creator8/8
  Demux6/2 -> Bus Creator8/2
  Demux6/9 -> Bus Creator8/9
  Demux6/5 -> Bus Creator8/5
  Demux6/3 -> Bus Creator8/3
  Demux6/7 -> Bus Creator8/7
  Demux6/1 -> Bus Creator8/1
  Demux6/6 -> Bus Creator8/6
  Demux6/10 -> Bus Creator8/10
  Bus Creator8/1 -> ?  "整车期望姿态"
  [F_N_flag] -> MATLAB Function2/2(flag)  "isFloating"
  Sum30/1 -> Mux4/5
  Sum32/1 -> Mux4/6
  Sum31/1 -> Mux4/7
  Constant22/1 -> [wz_torque]
  Sum24/1 -> Sum17/1
  Sum17/1 -> Product6/2
  Constant7/1 -> Sum17/2
  Constant12/1 -> Sum23/2
  Sum18/1 -> Sum23/1
  Sum23/1 -> Product5/2
  Sum11/1 -> [right_leg_forceD]
  Sum10/1 -> [left_leg_forceD]
  Cos/1 -> Product4/1
  Sum25/1 -> Cos/1
  [real_q] -> Sum25/1
  [real_rg_phi] -> Sum25/2
  [real_q] -> Sum26/1
  [real_lf_phi] -> Sum26/2
  Cos1/1 -> Product2/1
  Sum26/1 -> Cos1/1
  Product2/1 -> Sum11/1
  Bus Selector4/1 -> [real_roll]  "<roll>"
  Bus Selector4/2 -> [real_droll]  "<droll>"
  底盘roll&wroll/1 -> Bus Selector4/1
  Constant14/1 -> Sum27/2
  From61/1 -> Sum27/1
  Sum27/1 -> PID Controller9/1
  Constant4/1 -> Sum28/1
  Constant8/1 -> Sum29/2
  Sum29/1 -> Sum19/2
  Sum28/1 -> Sum8/2
  Constant18/1 -> Product3/1
  Constant25/1 -> Product3/2
  Product3/1 -> Product4/2, Product2/2
  [real_q] -> Sum30/2  "q"
  [real_lf_phi] -> Sum30/1  "lphi"
  [real_rg_phi] -> Sum31/1  "rphi"
  [real_rg_phi] -> Bus Creator3/2  "real_rg_phi"
  [real_q] -> Sum31/2  "q"
  [real_lf_dphi] -> Sum32/1  "ldphi"
  [real_dq] -> Sum32/2  "dq"
  [real_rg_dphi] -> Sum33/1  "rdphi"
  [real_dq] -> Sum33/2  "dq"
  Sum33/1 -> Mux4/8
  [chassis_az] -> Bus Creator/19  "chassis_az"
  底盘x轴加速度/1 -> [chassis_ax]
  底盘y轴加速度/1 -> [chassis_ay]
  [chassis_ax] -> Bus Creator/17  "chassis_ax"
  [chassis_ay] -> Bus Creator/18  "chassis_ay"
  [chassis_ay] -> 左腿离地检测2/4(底盘y轴加速度), 左腿离地检测1/4(底盘y轴加速度)
  [chassis_ax] -> 左腿离地检测2/3(底盘x轴加速度), 左腿离地检测1/3(底盘x轴加速度)
  [real_roll] -> 左腿离地检测2/2(roll), 左腿离地检测1/2(roll)
  [real_q] -> 左腿离地检测2/1(pitch), 左腿离地检测1/1(pitch)
  Constant16/1 -> Sum13/1
  Constant23/1 -> Sum13/2
  Sum13/1 -> MATLAB Function6/3(m)
  PID Controller9/1 -> Sum28/2, Sum29/1
  Zero-Order Hold/1 -> TorqueQ_left_leg/1
  [left_leg_forceD] -> ForceD_left_leg/1
  Zero-Order Hold2/1 -> TorqueQ_right_leg/1
  [right_leg_forceD] -> ForceD_right_leg/1
  Sum16/1 -> Torque_right_wheel/1
  Sum/1 -> Torque_left_wheel/1
  Discrete-Time Integrator1/1 -> [expt_int_xl]
  Memory/1 -> [F_N_flag]
  Constant1/1 -> Mux5/1

== system WBR_Simulator/腿建模 ==
  note: 这里准备了两种结构预设，直接替换即可
  TorqueQ_left_leg : Inport
  ForceD_left_leg : Inport  Port=2
  TorqueQ_right_leg : Inport  Port=3
  ForceD_right_leg : Inport  Port=4
  Bus Creator : BusCreator  Inputs=2
  Bus Creator1 : BusCreator  Inputs=4
  Bus Creator2 : BusCreator  Inputs=4
  Discrete Derivative : simulink/Discrete/Discrete Derivative  gainval=1.0  ICPrevScaledInput=0.0  OutMin=[]  OutMax=[]  OutDataType=fixdt(1, 16)  OutScaling=2^-10  DoSatur=off
  Discrete Derivative1 : simulink/Discrete/Discrete Derivative  gainval=1.0  ICPrevScaledInput=0.0  OutMin=[]  OutMax=[]  OutDataType=fixdt(1, 16)  OutScaling=2^-10  DoSatur=off
  Divide : Product  Inputs=*/
  Divide1 : Product  Inputs=*/
  Sum : Sum  Inputs=|-+
  Sum1 : Sum  Inputs=|-+
  串联腿 : Subsystem  Commented=on
      settings: PortSchema="{\"entries\":[{\"content\":{\"sides\":[{\"content\":{\"connectorIds\":[\"In1\",\"In2\",\"LConn1\",\"LConn2\"]},\"type\":\"ConnectorPlacement.EquallySpacedRectSide\",\"uuid\":\"c09ee776-e3b2-4671-a777-05334f39d539\"},{\"content\":{\"connectorIds\":[\"Out1\",\"Out2\",\"Out3\",\"Out4\",\"RConn1\",\"RConn2\"],\"side\":\"RIGHT\"},\"type\":\"ConnectorPlacement.EquallySpacedRectSide\",\"uuid\":\"c9a818ad-ac1f-44fd-9e7e-fd9bd89e73b7\"},{\"content\":{\"side\":\"TOP\"},\"type\":\"ConnectorPlacement.EquallySpacedRectSide\",\"uuid\":\"95a2c650-09cf-4f49-b028-1c47e21ec5e1\"},{\"content\":{\"connectorIds\":[\"Out5\"],\"side\":\"BOTTOM\"},\"type\":\"ConnectorPlacement.EquallySpacedRectSide\",\"uuid\":\"11dd9153-b274-4998-a336-51cb62729214\"}]},\"type\":\"ConnectorPlacement.EquallySpacedConnector\",\"uuid\":\"3d8489c2-6bc1-4528-9c85-2076b5b81c0c\"}],\"packageUris\":[\"http://schema.mathworks.com/mf0/Connector/R2020b\"],\"version\":\"1.0\"}"
  并联腿 : Subsystem  Commented=on
      settings: PortSchema="{\"entries\":[{\"content\":{\"sides\":[{\"content\":{\"connectorIds\":[\"In1\",\"In2\",\"LConn1\",\"LConn2\"]},\"type\":\"ConnectorPlacement.EquallySpacedRectSide\",\"uuid\":\"c09ee776-e3b2-4671-a777-05334f39d539\"},{\"content\":{\"connectorIds\":[\"Out1\",\"Out2\",\"Out3\",\"Out4\",\"RConn1\",\"RConn2\"],\"side\":\"RIGHT\"},\"type\":\"ConnectorPlacement.EquallySpacedRectSide\",\"uuid\":\"c9a818ad-ac1f-44fd-9e7e-fd9bd89e73b7\"},{\"content\":{\"side\":\"TOP\"},\"type\":\"ConnectorPlacement.EquallySpacedRectSide\",\"uuid\":\"95a2c650-09cf-4f49-b028-1c47e21ec5e1\"},{\"content\":{\"connectorIds\":[\"Out5\"],\"side\":\"BOTTOM\"},\"type\":\"ConnectorPlacement.EquallySpacedRectSide\",\"uuid\":\"11dd9153-b274-4998-a336-51cb62729214\"}]},\"type\":\"ConnectorPlacement.EquallySpacedConnector\",\"uuid\":\"3d8489c2-6bc1-4528-9c85-2076b5b81c0c\"}],\"packageUris\":[\"http://schema.mathworks.com/mf0/Connector/R2020b\"],\"version\":\"1.0\"}"
  并联腿1 : Subsystem
      settings: PortSchema="{\"entries\":[{\"content\":{\"sides\":[{\"content\":{\"connectorIds\":[\"In1\",\"In2\",\"LConn1\",\"LConn2\"]},\"type\":\"ConnectorPlacement.EquallySpacedRectSide\",\"uuid\":\"c09ee776-e3b2-4671-a777-05334f39d539\"},{\"content\":{\"connectorIds\":[\"Out1\",\"Out2\",\"Out3\",\"Out4\",\"RConn1\",\"RConn2\"],\"side\":\"RIGHT\"},\"type\":\"ConnectorPlacement.EquallySpacedRectSide\",\"uuid\":\"c9a818ad-ac1f-44fd-9e7e-fd9bd89e73b7\"},{\"content\":{\"side\":\"TOP\"},\"type\":\"ConnectorPlacement.EquallySpacedRectSide\",\"uuid\":\"95a2c650-09cf-4f49-b028-1c47e21ec5e1\"},{\"content\":{\"connectorIds\":[\"Out5\"],\"side\":\"BOTTOM\"},\"type\":\"ConnectorPlacement.EquallySpacedRectSide\",\"uuid\":\"11dd9153-b274-4998-a336-51cb62729214\"}]},\"type\":\"ConnectorPlacement.EquallySpacedConnector\",\"uuid\":\"3d8489c2-6bc1-4528-9c85-2076b5b81c0c\"}],\"packageUris\":[\"http://schema.mathworks.com/mf0/Connector/R2020b\"],\"version\":\"1.0\"}"
  并联腿2 : Subsystem
      settings: PortSchema="{\"entries\":[{\"content\":{\"sides\":[{\"content\":{\"connectorIds\":[\"In1\",\"In2\",\"LConn1\",\"LConn2\"]},\"type\":\"ConnectorPlacement.EquallySpacedRectSide\",\"uuid\":\"c09ee776-e3b2-4671-a777-05334f39d539\"},{\"content\":{\"connectorIds\":[\"Out1\",\"Out2\",\"Out3\",\"Out4\",\"RConn1\",\"RConn2\"],\"side\":\"RIGHT\"},\"type\":\"ConnectorPlacement.EquallySpacedRectSide\",\"uuid\":\"c9a818ad-ac1f-44fd-9e7e-fd9bd89e73b7\"},{\"content\":{\"side\":\"TOP\"},\"type\":\"ConnectorPlacement.EquallySpacedRectSide\",\"uuid\":\"95a2c650-09cf-4f49-b028-1c47e21ec5e1\"},{\"content\":{\"connectorIds\":[\"Out5\"],\"side\":\"BOTTOM\"},\"type\":\"ConnectorPlacement.EquallySpacedRectSide\",\"uuid\":\"11dd9153-b274-4998-a336-51cb62729214\"}]},\"type\":\"ConnectorPlacement.EquallySpacedConnector\",\"uuid\":\"3d8489c2-6bc1-4528-9c85-2076b5b81c0c\"}],\"packageUris\":[\"http://schema.mathworks.com/mf0/Connector/R2020b\"],\"version\":\"1.0\"}"
  chassis_right_side_frame : PMIOPort  Side=Right
  chassis_left_side_frame : PMIOPort  Port=2  Side=Right
  right_wheel_frame : PMIOPort  Port=3  Side=Right
  left_wheel_frame : PMIOPort  Port=4  Side=Right
  底盘地面碰撞 : PMIOPort  Port=5  Side=Right
  底盘飞坡碰撞 : PMIOPort  Port=6  Side=Right
  left_leg : Outport
  right_leg : Outport  Port=2
  valid_torque : Outport  Port=3
  wires:
  Bus Creator1/1 -> left_leg/1  "left_leg"
  ForceD_left_leg/1 -> 并联腿1/2(设定径向力)
  TorqueQ_left_leg/1 -> 并联腿1/1(设定切向力矩)
  并联腿1/2(L_0) -> Discrete Derivative1/1, Bus Creator1/2, Divide/2  "real_L"
  并联腿1/1(phi_0) -> Bus Creator1/1  "real_phi"
  Divide/1 -> Bus Creator1/3  "real_omega"
  ForceD_right_leg/1 -> 并联腿2/2(设定径向力)
  并联腿2/1(phi_0) -> Bus Creator2/1  "real_phi"
  Divide1/1 -> Bus Creator2/3  "real_omega"
  TorqueQ_right_leg/1 -> 并联腿2/1(设定切向力矩)
  Bus Creator2/1 -> right_leg/1  "right_leg"
  并联腿1/3(real_vq) -> Divide/1
  并联腿2/3(real_vq) -> Divide1/1
  并联腿1/4(real_vd) -> Bus Creator1/4, Sum/2  "real_dl"
  并联腿2/2(L_0) -> Discrete Derivative/1, Bus Creator2/2, Divide1/2  "real_L"
  Discrete Derivative1/1 -> Sum/1  "real_dl"
  Sum/1 -> ?  "error_d1"
  并联腿2/4(real_vd) -> Bus Creator2/4, Sum1/2  "real_dl"
  Discrete Derivative/1 -> Sum1/1  "real_dl"
  Sum1/1 -> ?  "error_d2"
  并联腿1/5(valid_tqd) -> Bus Creator/1  "左腿"
  并联腿2/5(valid_tqd) -> Bus Creator/2  "右腿"
  Bus Creator/1 -> valid_torque/1  "腿真实有效力"
  connections:
  并联腿1/LConn2 -- left_wheel_frame/RConn1
  并联腿1/LConn1 -- chassis_left_side_frame/RConn1
  并联腿2/LConn2 -- right_wheel_frame/RConn1
  并联腿2/LConn1 -- chassis_right_side_frame/RConn1
  并联腿2/RConn1 -- 底盘地面碰撞/RConn1 -- 并联腿1/RConn1
  并联腿2/RConn2 -- 底盘飞坡碰撞/RConn1 -- 并联腿1/RConn2
